simulink model "rfdac_lo_jitter_link_budget"  (R2024a)
settings: Solver=FixedStepDiscrete  StartTime=0.0  StopTime=p.Stop_Time  FixedStep=p.Frame_Period  RelTol=1e-3
PostLoadFcn:
  | addpath(fileparts(get_param('rfdac_lo_jitter_link_budget','FileName'))); setup_rfdac_project;
  | update_rfdac_rx_equalizer_model('rfdac_lo_jitter_link_budget');
  | update_rfdac_lo_amplitude_model('rfdac_lo_jitter_link_budget');
InitFcn:
  | rfdac_model_init;
values from neighbouring files (symbols this model uses):
  cfg = rfdac_default_config()    [init_rfdac_identification.m]    (also in init_rfdac_model.m; run_rfdac_simulation.m = evalin('base','cfg'))
  p = evalin('base','p')    [run_rfdac_simulation.m]
Description:
  | RF TX target-EVM calibration, four-phase LO quadrature imbalance and timing jitter.
settings Model: Creator=Admin  LastModifiedBy=Admin
settings DataIOCC: SaveOutput=off  SignalLogging=off  SaveTime=off

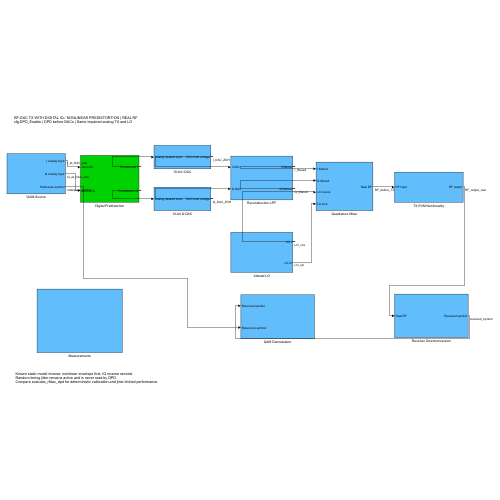
[thumbnail: Simulink's stored preview of the top-level diagram]
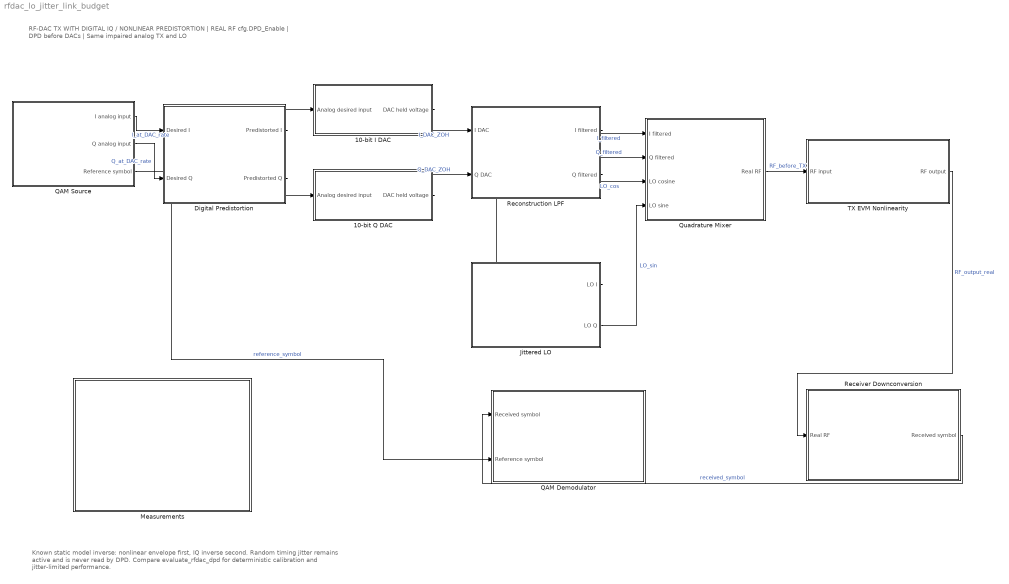
== system rfdac_lo_jitter_link_budget ==
  note: RF-DAC TX WITH DIGITAL IQ / NONLINEAR PREDISTORTION | REAL RF
      | cfg.DPD_Enable | DPD before DACs | Same impaired analog TX and LO
  note: Known static model inverse: nonlinear envelope first, IQ inverse second.
      | Random timing jitter remains active and is never read by DPD.
      | Compare evaluate_rfdac_dpd for deterministic calibration and jitter-limited performance.
  10-bit I DAC : Subsystem
  10-bit Q DAC : Subsystem
  Digital Predistortion : Subsystem  Tag=rfdac_dpd_v7
  Jittered LO : Subsystem
  Measurements : Subsystem
  QAM Demodulator : Subsystem
  QAM Source : Subsystem
  Quadrature Mixer : Subsystem
  Receiver Downconversion : Subsystem
  Reconstruction LPF : Subsystem
  TX EVM Nonlinearity : Subsystem  Tag=rfdac_evm_v2
  wires:
  10-bit I DAC/1(DAC held voltage) -> Reconstruction LPF/1(I DAC)  "I_DAC_ZOH"
  10-bit Q DAC/1(DAC held voltage) -> Reconstruction LPF/2(Q DAC)  "Q_DAC_ZOH"
  Reconstruction LPF/1(I filtered) -> Quadrature Mixer/1(I filtered)  "I_filtered"
  Reconstruction LPF/2(Q filtered) -> Quadrature Mixer/2(Q filtered)  "Q_filtered"
  Jittered LO/1(LO I) -> Quadrature Mixer/3(LO cosine)  "LO_cos"
  Jittered LO/2(LO Q) -> Quadrature Mixer/4(LO sine)  "LO_sin"
  Quadrature Mixer/1(Real RF) -> TX EVM Nonlinearity/1(RF input)  "RF_before_TX"
  TX EVM Nonlinearity/1(RF output) -> Receiver Downconversion/1(Real RF)  "RF_output_real"
  Receiver Downconversion/1(Received symbol) -> QAM Demodulator/1(Received symbol)  "received_symbol"
  QAM Source/3(Reference symbol) -> QAM Demodulator/2(Reference symbol)  "reference_symbol"
  QAM Source/1(I analog input) -> Digital Predistortion/1(Desired I)  "I_at_DAC_rate"
  QAM Source/2(Q analog input) -> Digital Predistortion/2(Desired Q)  "Q_at_DAC_rate"
  Digital Predistortion/1(Predistorted I) -> 10-bit I DAC/1(Analog desired input)
  Digital Predistortion/2(Predistorted Q) -> 10-bit Q DAC/1(Analog desired input)

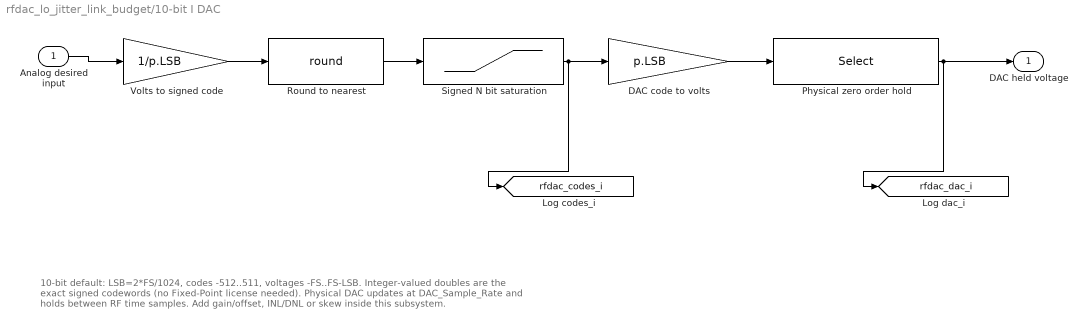
== system rfdac_lo_jitter_link_budget/10-bit I DAC ==
  note: 10-bit default: LSB=2*FS/1024, codes -512..511, voltages -FS..FS-LSB.
      | Integer-valued doubles are the exact signed codewords (no Fixed-Point license needed).
      | Physical DAC updates at DAC_Sample_Rate and holds between RF time samples.
      | Add gain/offset, INL/DNL or skew inside this subsystem.
  Analog desired input : Inport
  DAC code to volts : Gain  Gain=p.LSB
  Physical zero order hold : Selector  InputPortWidth=p.DAC_Samples_Per_Symbol  IndexOptions=Index vector (dialog)  Indices=p.DAC_Hold_Indices  OutputSizes=1
  Round to nearest : Rounding  Operator=round
  Signed N bit saturation : Saturate  UpperLimit=p.Max_Code  LowerLimit=p.Min_Code
  Volts to signed code : Gain  Gain=1/p.LSB
  DAC held voltage : Outport
  tag scope: rfdac_codes_i=global, rfdac_dac_i=global
  wires:
  Analog desired input/1 -> Volts to signed code/1
  Volts to signed code/1 -> Round to nearest/1
  Round to nearest/1 -> Signed N bit saturation/1
  Signed N bit saturation/1 -> DAC code to volts/1, [rfdac_codes_i]
  DAC code to volts/1 -> Physical zero order hold/1
  Physical zero order hold/1 -> DAC held voltage/1, [rfdac_dac_i]

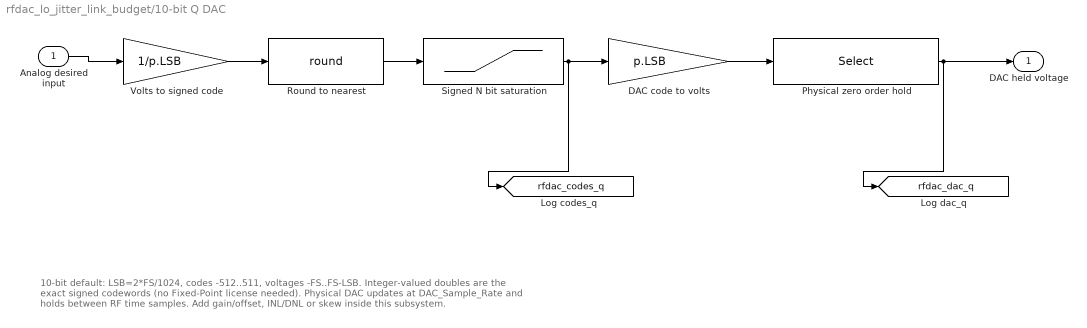
== system rfdac_lo_jitter_link_budget/10-bit Q DAC ==
  note: 10-bit default: LSB=2*FS/1024, codes -512..511, voltages -FS..FS-LSB.
      | Integer-valued doubles are the exact signed codewords (no Fixed-Point license needed).
      | Physical DAC updates at DAC_Sample_Rate and holds between RF time samples.
      | Add gain/offset, INL/DNL or skew inside this subsystem.
  Analog desired input : Inport
  DAC code to volts : Gain  Gain=p.LSB
  Physical zero order hold : Selector  InputPortWidth=p.DAC_Samples_Per_Symbol  IndexOptions=Index vector (dialog)  Indices=p.DAC_Hold_Indices  OutputSizes=1
  Round to nearest : Rounding  Operator=round
  Signed N bit saturation : Saturate  UpperLimit=p.Max_Code  LowerLimit=p.Min_Code
  Volts to signed code : Gain  Gain=1/p.LSB
  DAC held voltage : Outport
  tag scope: rfdac_codes_q=global, rfdac_dac_q=global
  wires:
  Analog desired input/1 -> Volts to signed code/1
  Volts to signed code/1 -> Round to nearest/1
  Round to nearest/1 -> Signed N bit saturation/1
  Signed N bit saturation/1 -> DAC code to volts/1, [rfdac_codes_q]
  DAC code to volts/1 -> Physical zero order hold/1
  Physical zero order hold/1 -> DAC held voltage/1, [rfdac_dac_q]

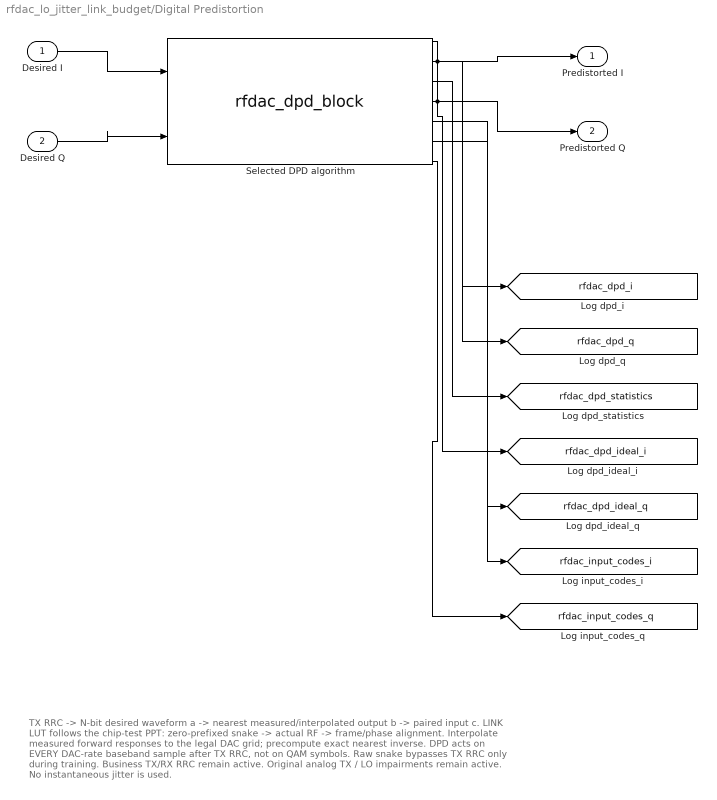
== system rfdac_lo_jitter_link_budget/Digital Predistortion ==
  note: TX RRC -> N-bit desired waveform a -> nearest measured/interpolated output b -> paired input c.
      | LINK LUT follows the chip-test PPT: zero-prefixed snake -> actual RF -> frame/phase alignment.
      | Interpolate measured forward responses to the legal DAC grid; precompute exact nearest inverse.
      | DPD acts on EVERY DAC-rate baseband sample after TX RRC, not on QAM symbols.
      | Raw snake bypasses TX RRC only during training. Business TX/RX RRC remain active.
      | Original analog TX / LO impairments remain active. No instantaneous jitter is used.
  Desired I : Inport
  Desired Q : Inport  Port=2
  Selected DPD algorithm : M-S-Function  FunctionName=rfdac_dpd_block  Parameters=p.DPD_Runtime,p.DAC_Samples_Per_Symbol
  Predistorted I : Outport
  Predistorted Q : Outport  Port=2
  tag scope: rfdac_dpd_i=global, rfdac_dpd_ideal_i=global, rfdac_dpd_ideal_q=global, rfdac_dpd_q=global, rfdac_dpd_statistics=global, rfdac_input_codes_i=global, rfdac_input_codes_q=global
  wires:
  Desired I/1 -> Selected DPD algorithm/1
  Desired Q/1 -> Selected DPD algorithm/2
  Selected DPD algorithm/1 -> Predistorted I/1, [rfdac_dpd_i]
  Selected DPD algorithm/2 -> Predistorted Q/1, [rfdac_dpd_q]
  Selected DPD algorithm/3 -> [rfdac_dpd_statistics]
  Selected DPD algorithm/4 -> [rfdac_dpd_ideal_i]
  Selected DPD algorithm/5 -> [rfdac_dpd_ideal_q]
  Selected DPD algorithm/6 -> [rfdac_input_codes_i]
  Selected DPD algorithm/7 -> [rfdac_input_codes_q]

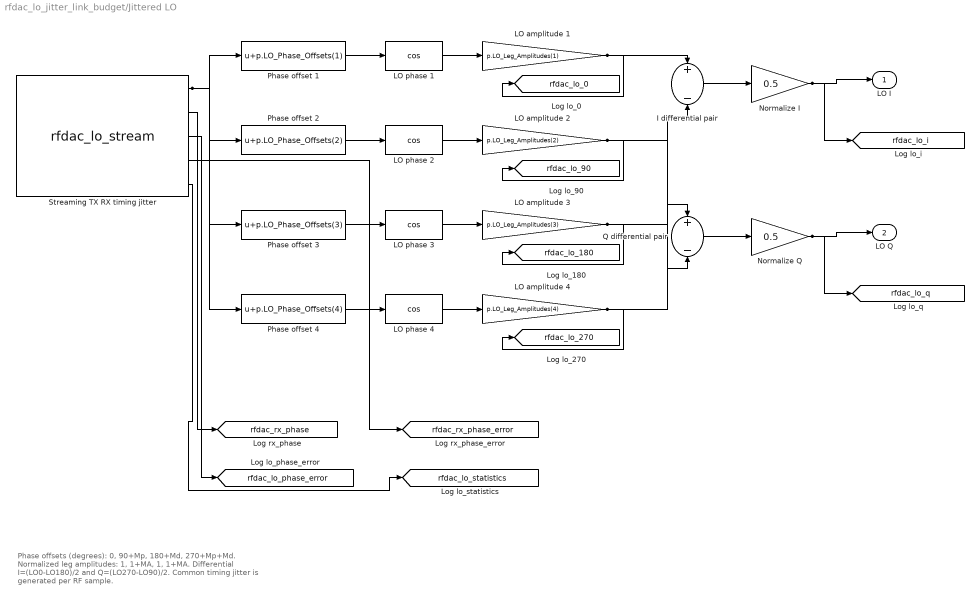
== system rfdac_lo_jitter_link_budget/Jittered LO ==
  note: Phase offsets (degrees): 0, 90+Mp, 180+Md, 270+Mp+Md.
      | Normalized leg amplitudes: 1, 1+MA, 1, 1+MA.
      | Differential I=(LO0-LO180)/2 and Q=(LO270-LO90)/2.
      | Common timing jitter is generated per RF sample.
  I differential pair : Sum  Inputs=+-
  LO amplitude 1 : Gain  Tag=rfdac_lo_leg_amplitude_v1  Gain=p.LO_Leg_Amplitudes(1)
  LO amplitude 2 : Gain  Tag=rfdac_lo_leg_amplitude_v1  Gain=p.LO_Leg_Amplitudes(2)
  LO amplitude 3 : Gain  Tag=rfdac_lo_leg_amplitude_v1  Gain=p.LO_Leg_Amplitudes(3)
  LO amplitude 4 : Gain  Tag=rfdac_lo_leg_amplitude_v1  Gain=p.LO_Leg_Amplitudes(4)
  LO phase {1..4} (4 alike) : Trigonometry  Operator=cos
  Normalize I : Gain  Gain=0.5
  Normalize Q : Gain  Gain=0.5
  Phase offset 1 : Bias  Bias=p.LO_Phase_Offsets(1)  SaturateOnIntegerOverflow=off
  Phase offset 2 : Bias  Bias=p.LO_Phase_Offsets(2)  SaturateOnIntegerOverflow=off
  Phase offset 3 : Bias  Bias=p.LO_Phase_Offsets(3)  SaturateOnIntegerOverflow=off
  Phase offset 4 : Bias  Bias=p.LO_Phase_Offsets(4)  SaturateOnIntegerOverflow=off
  Q differential pair : Sum  Inputs=+-
  Streaming TX RX timing jitter : M-S-Function  FunctionName=rfdac_lo_stream  Parameters=cfg,p.Samples_Per_Symbol
  LO I : Outport
  LO Q : Outport  Port=2
  tag scope: rfdac_lo_0=global, rfdac_lo_180=global, rfdac_lo_270=global, rfdac_lo_90=global, rfdac_lo_i=global, rfdac_lo_phase_error=global, rfdac_lo_q=global, rfdac_lo_statistics=global, rfdac_rx_phase=global, rfdac_rx_phase_error=global
  wires:
  Streaming TX RX timing jitter/1 -> Phase offset 1/1, Phase offset 2/1, Phase offset 3/1, Phase offset 4/1
  Phase offset 1/1 -> LO phase 1/1
  Phase offset 2/1 -> LO phase 2/1
  Phase offset 3/1 -> LO phase 3/1
  Phase offset 4/1 -> LO phase 4/1
  I differential pair/1 -> Normalize I/1
  Q differential pair/1 -> Normalize Q/1
  Normalize I/1 -> LO I/1, [rfdac_lo_i]
  Normalize Q/1 -> LO Q/1, [rfdac_lo_q]
  Streaming TX RX timing jitter/2 -> [rfdac_rx_phase]
  Streaming TX RX timing jitter/3 -> [rfdac_lo_phase_error]
  Streaming TX RX timing jitter/4 -> [rfdac_rx_phase_error]
  Streaming TX RX timing jitter/5 -> [rfdac_lo_statistics]
  LO phase 1/1 -> LO amplitude 1/1
  LO amplitude 1/1 -> [rfdac_lo_0], I differential pair/1
  LO phase 2/1 -> LO amplitude 2/1
  LO amplitude 2/1 -> [rfdac_lo_90], Q differential pair/2
  LO phase 3/1 -> LO amplitude 3/1
  LO amplitude 3/1 -> [rfdac_lo_180], I differential pair/2
  LO phase 4/1 -> LO amplitude 4/1
  LO amplitude 4/1 -> [rfdac_lo_270], Q differential pair/1

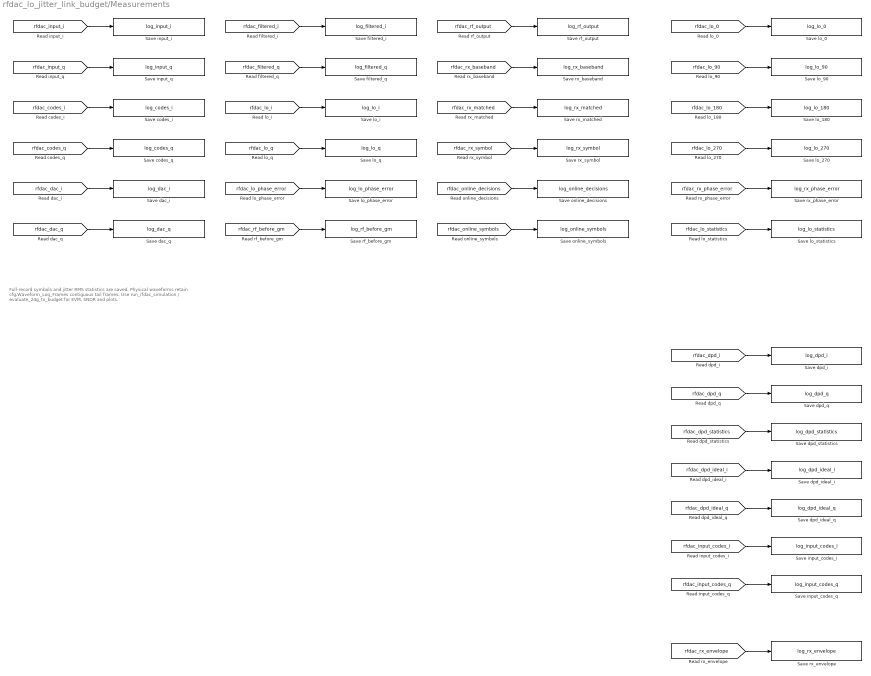
== system rfdac_lo_jitter_link_budget/Measurements ==
  note: Full-record symbols and jitter RMS statistics are saved.
      | Physical waveforms retain cfg.Waveform_Log_Frames contiguous tail frames.
      | Use run_rfdac_simulation / evaluate_24g_tx_budget for EVM, SNDR and plots.
  Save codes_i : ToWorkspace  VariableName=log_codes_i  SaveFormat=Structure With Time  SampleTime=-1
      settings: MaxDataPoints=cfg.Waveform_Log_Frames
  Save codes_q : ToWorkspace  VariableName=log_codes_q  SaveFormat=Structure With Time  SampleTime=-1
      settings: MaxDataPoints=cfg.Waveform_Log_Frames
  Save dac_i : ToWorkspace  VariableName=log_dac_i  SaveFormat=Structure With Time  SampleTime=-1
      settings: MaxDataPoints=cfg.Waveform_Log_Frames
  Save dac_q : ToWorkspace  VariableName=log_dac_q  SaveFormat=Structure With Time  SampleTime=-1
      settings: MaxDataPoints=cfg.Waveform_Log_Frames
  Save dpd_i : ToWorkspace  VariableName=log_dpd_i  SaveFormat=Structure With Time  SampleTime=-1
      settings: MaxDataPoints=cfg.Waveform_Log_Frames
  Save dpd_ideal_i : ToWorkspace  VariableName=log_dpd_ideal_i  SaveFormat=Structure With Time  SampleTime=-1
      settings: MaxDataPoints=cfg.Waveform_Log_Frames
  Save dpd_ideal_q : ToWorkspace  VariableName=log_dpd_ideal_q  SaveFormat=Structure With Time  SampleTime=-1
      settings: MaxDataPoints=cfg.Waveform_Log_Frames
  Save dpd_q : ToWorkspace  VariableName=log_dpd_q  SaveFormat=Structure With Time  SampleTime=-1
      settings: MaxDataPoints=cfg.Waveform_Log_Frames
  Save dpd_statistics : ToWorkspace  VariableName=log_dpd_statistics  SaveFormat=Structure With Time  SampleTime=-1
  Save filtered_i : ToWorkspace  VariableName=log_filtered_i  SaveFormat=Structure With Time  SampleTime=-1
      settings: MaxDataPoints=cfg.Waveform_Log_Frames
  Save filtered_q : ToWorkspace  VariableName=log_filtered_q  SaveFormat=Structure With Time  SampleTime=-1
      settings: MaxDataPoints=cfg.Waveform_Log_Frames
  Save input_codes_i : ToWorkspace  VariableName=log_input_codes_i  SaveFormat=Structure With Time  SampleTime=-1
      settings: MaxDataPoints=cfg.Waveform_Log_Frames
  Save input_codes_q : ToWorkspace  VariableName=log_input_codes_q  SaveFormat=Structure With Time  SampleTime=-1
      settings: MaxDataPoints=cfg.Waveform_Log_Frames
  Save input_i : ToWorkspace  VariableName=log_input_i  SaveFormat=Structure With Time  SampleTime=-1
      settings: MaxDataPoints=cfg.Waveform_Log_Frames
  Save input_q : ToWorkspace  VariableName=log_input_q  SaveFormat=Structure With Time  SampleTime=-1
      settings: MaxDataPoints=cfg.Waveform_Log_Frames
  Save lo_0 : ToWorkspace  VariableName=log_lo_0  SaveFormat=Structure With Time  SampleTime=-1
      settings: MaxDataPoints=cfg.Waveform_Log_Frames
  Save lo_180 : ToWorkspace  VariableName=log_lo_180  SaveFormat=Structure With Time  SampleTime=-1
      settings: MaxDataPoints=cfg.Waveform_Log_Frames
  Save lo_270 : ToWorkspace  VariableName=log_lo_270  SaveFormat=Structure With Time  SampleTime=-1
      settings: MaxDataPoints=cfg.Waveform_Log_Frames
  Save lo_90 : ToWorkspace  VariableName=log_lo_90  SaveFormat=Structure With Time  SampleTime=-1
      settings: MaxDataPoints=cfg.Waveform_Log_Frames
  Save lo_i : ToWorkspace  VariableName=log_lo_i  SaveFormat=Structure With Time  SampleTime=-1
      settings: MaxDataPoints=cfg.Waveform_Log_Frames
  Save lo_phase_error : ToWorkspace  VariableName=log_lo_phase_error  SaveFormat=Structure With Time  SampleTime=-1
      settings: MaxDataPoints=cfg.Waveform_Log_Frames
  Save lo_q : ToWorkspace  VariableName=log_lo_q  SaveFormat=Structure With Time  SampleTime=-1
      settings: MaxDataPoints=cfg.Waveform_Log_Frames
  Save lo_statistics : ToWorkspace  VariableName=log_lo_statistics  SaveFormat=Structure With Time  SampleTime=-1
  Save online_decisions : ToWorkspace  VariableName=log_online_decisions  SaveFormat=Structure With Time  SampleTime=-1
  Save online_symbols : ToWorkspace  VariableName=log_online_symbols  SaveFormat=Structure With Time  SampleTime=-1
  Save rf_before_gm : ToWorkspace  VariableName=log_rf_before_gm  SaveFormat=Structure With Time  SampleTime=-1
      settings: MaxDataPoints=cfg.Waveform_Log_Frames
  Save rf_output : ToWorkspace  VariableName=log_rf_output  SaveFormat=Structure With Time  SampleTime=-1
      settings: MaxDataPoints=cfg.Waveform_Log_Frames
  Save rx_baseband : ToWorkspace  VariableName=log_rx_baseband  SaveFormat=Structure With Time  SampleTime=-1
      settings: MaxDataPoints=cfg.Waveform_Log_Frames
  Save rx_envelope : ToWorkspace  VariableName=log_rx_envelope  SaveFormat=Structure With Time  SampleTime=-1
      settings: MaxDataPoints=p.Observation_Log_Frames
  Save rx_matched : ToWorkspace  VariableName=log_rx_matched  SaveFormat=Structure With Time  SampleTime=-1
      settings: MaxDataPoints=cfg.Waveform_Log_Frames
  Save rx_phase_error : ToWorkspace  VariableName=log_rx_phase_error  SaveFormat=Structure With Time  SampleTime=-1
      settings: MaxDataPoints=cfg.Waveform_Log_Frames
  Save rx_symbol : ToWorkspace  VariableName=log_rx_symbol  SaveFormat=Structure With Time  SampleTime=-1
  wires:
  [rfdac_input_i] -> Save input_i/1
  [rfdac_input_q] -> Save input_q/1
  [rfdac_codes_i] -> Save codes_i/1
  [rfdac_codes_q] -> Save codes_q/1
  [rfdac_dac_i] -> Save dac_i/1
  [rfdac_dac_q] -> Save dac_q/1
  [rfdac_filtered_i] -> Save filtered_i/1
  [rfdac_filtered_q] -> Save filtered_q/1
  [rfdac_lo_i] -> Save lo_i/1
  [rfdac_lo_q] -> Save lo_q/1
  [rfdac_lo_phase_error] -> Save lo_phase_error/1
  [rfdac_rf_before_gm] -> Save rf_before_gm/1
  [rfdac_rf_output] -> Save rf_output/1
  [rfdac_rx_baseband] -> Save rx_baseband/1
  [rfdac_rx_matched] -> Save rx_matched/1
  [rfdac_rx_symbol] -> Save rx_symbol/1
  [rfdac_online_decisions] -> Save online_decisions/1
  [rfdac_online_symbols] -> Save online_symbols/1
  [rfdac_lo_0] -> Save lo_0/1
  [rfdac_lo_90] -> Save lo_90/1
  [rfdac_lo_180] -> Save lo_180/1
  [rfdac_lo_270] -> Save lo_270/1
  [rfdac_rx_phase_error] -> Save rx_phase_error/1
  [rfdac_lo_statistics] -> Save lo_statistics/1
  [rfdac_dpd_i] -> Save dpd_i/1
  [rfdac_dpd_q] -> Save dpd_q/1
  [rfdac_dpd_statistics] -> Save dpd_statistics/1
  [rfdac_dpd_ideal_i] -> Save dpd_ideal_i/1
  [rfdac_dpd_ideal_q] -> Save dpd_ideal_q/1
  [rfdac_input_codes_i] -> Save input_codes_i/1
  [rfdac_input_codes_q] -> Save input_codes_q/1
  [rfdac_rx_envelope] -> Save rx_envelope/1

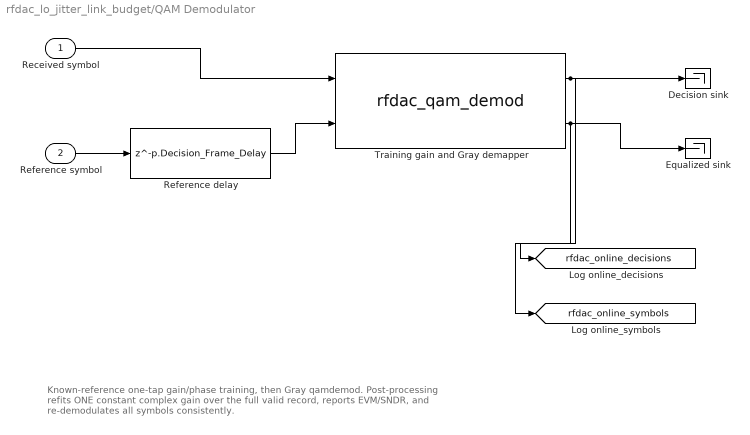
== system rfdac_lo_jitter_link_budget/QAM Demodulator ==
  note: Known-reference one-tap gain/phase training, then Gray qamdemod.
      | Post-processing refits ONE constant complex gain over the full valid record,
      | reports EVM/SNDR, and re-demodulates all symbols consistently.
  Received symbol : Inport
  Reference symbol : Inport  Port=2
  Decision sink : Terminator
  Equalized sink : Terminator
  Reference delay : Delay  DelayLength=p.Decision_Frame_Delay
  Training gain and Gray demapper : M-S-Function  FunctionName=rfdac_qam_demod  Parameters=cfg.QAM_Order
  tag scope: rfdac_online_decisions=global, rfdac_online_symbols=global
  wires:
  Received symbol/1 -> Training gain and Gray demapper/1
  Reference symbol/1 -> Reference delay/1
  Reference delay/1 -> Training gain and Gray demapper/2
  Training gain and Gray demapper/1 -> Decision sink/1, [rfdac_online_decisions]
  Training gain and Gray demapper/2 -> Equalized sink/1, [rfdac_online_symbols]

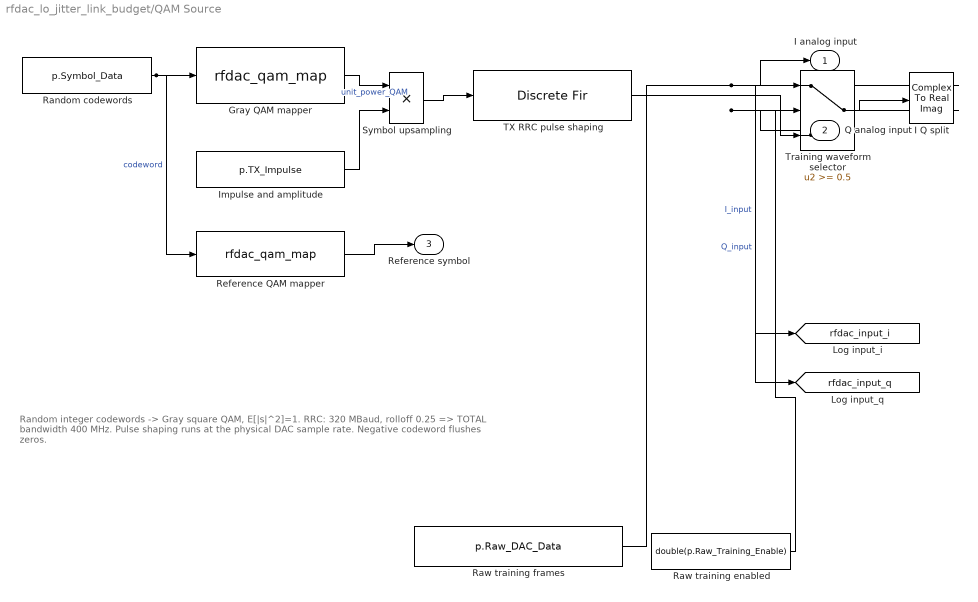
== system rfdac_lo_jitter_link_budget/QAM Source ==
  note: Random integer codewords -> Gray square QAM, E[|s|^2]=1.
      | RRC: 320 MBaud, rolloff 0.25 => TOTAL bandwidth 400 MHz.
      | Pulse shaping runs at the physical DAC sample rate. Negative codeword flushes zeros.
  Gray QAM mapper : M-S-Function  FunctionName=rfdac_qam_map  Parameters=p.Source_Constellation
  I Q split : ComplexToRealImag
  Impulse and amplitude : Constant  Value=p.TX_Impulse
  Random codewords : FromWorkspace  VariableName=p.Symbol_Data  SampleTime=p.Frame_Period  Interpolate=off  OutputAfterFinalValue=Holding final value
  Raw training enabled : Constant  Value=double(p.Raw_Training_Enable)
  Raw training frames : FromWorkspace  VariableName=p.Raw_DAC_Data  SampleTime=p.Frame_Period  Interpolate=off  OutputAfterFinalValue=Holding final value
  Reference QAM mapper : M-S-Function  FunctionName=rfdac_qam_map  Parameters=p.Constellation
  Symbol upsampling : Product
  TX RRC pulse shaping : DiscreteFir  Coefficients=p.RRC  InputProcessing=Columns as channels (frame based)
  Training waveform selector : Switch  Threshold=0.5  SaturateOnIntegerOverflow=off  InputSameDT=off
  I analog input : Outport
  Q analog input : Outport  Port=2
  Reference symbol : Outport  Port=3
  tag scope: rfdac_input_i=global, rfdac_input_q=global
  wires:
  Random codewords/1 -> Gray QAM mapper/1, Reference QAM mapper/1  "codeword"
  Gray QAM mapper/1 -> Symbol upsampling/1  "unit_power_QAM"
  Impulse and amplitude/1 -> Symbol upsampling/2
  Symbol upsampling/1 -> TX RRC pulse shaping/1
  I Q split/1 -> I analog input/1, [rfdac_input_i]  "I_input"
  I Q split/2 -> Q analog input/1, [rfdac_input_q]  "Q_input"
  Reference QAM mapper/1 -> Reference symbol/1
  Raw training frames/1 -> Training waveform selector/1
  Raw training enabled/1 -> Training waveform selector/2
  TX RRC pulse shaping/1 -> Training waveform selector/3
  Training waveform selector/1 -> I Q split/1

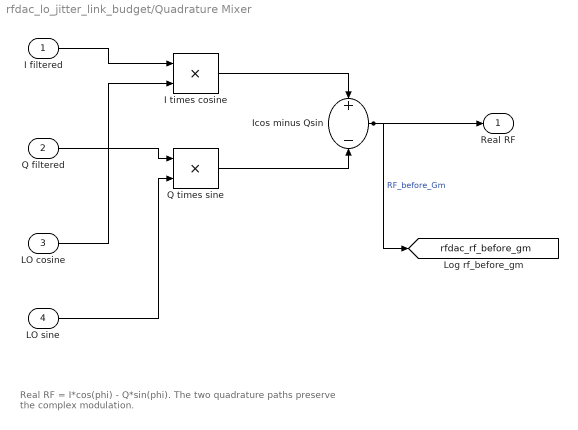
== system rfdac_lo_jitter_link_budget/Quadrature Mixer ==
  note: Real RF = I*cos(phi) - Q*sin(phi).
      | The two quadrature paths preserve the complex modulation.
  I filtered : Inport
  Q filtered : Inport  Port=2
  LO cosine : Inport  Port=3
  LO sine : Inport  Port=4
  I times cosine : Product
  Icos minus Qsin : Sum  Inputs=+-
  Q times sine : Product
  Real RF : Outport
  tag scope: rfdac_rf_before_gm=global
  wires:
  I filtered/1 -> I times cosine/1
  LO cosine/1 -> I times cosine/2
  Q filtered/1 -> Q times sine/1
  LO sine/1 -> Q times sine/2
  I times cosine/1 -> Icos minus Qsin/1
  Q times sine/1 -> Icos minus Qsin/2
  Icos minus Qsin/1 -> Real RF/1, [rfdac_rf_before_gm]  "RF_before_Gm"

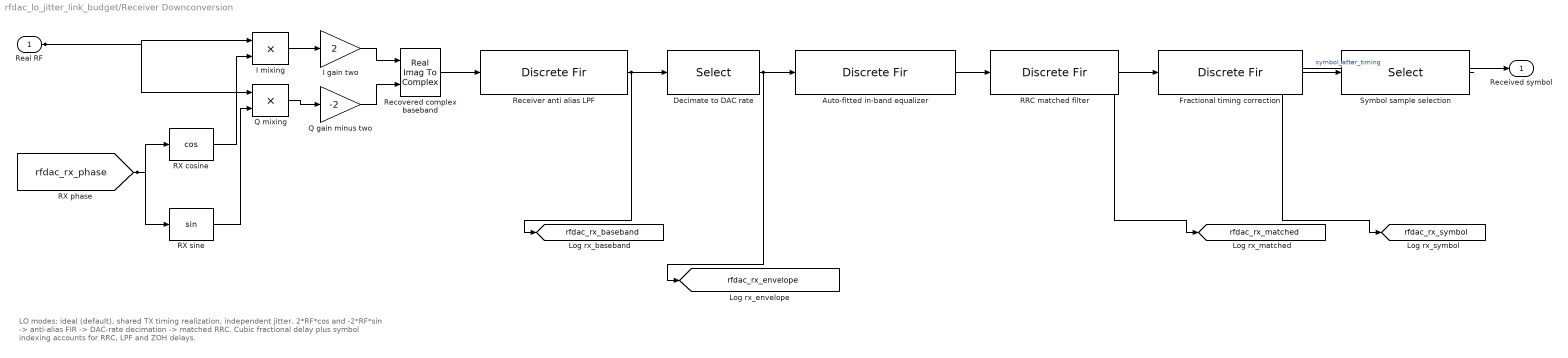
== system rfdac_lo_jitter_link_budget/Receiver Downconversion ==
  note: LO modes: ideal (default), shared TX timing realization, independent jitter.
      | 2*RF*cos and -2*RF*sin -> anti-alias FIR -> DAC-rate decimation -> matched RRC.
      | Cubic fractional delay plus symbol indexing accounts for RRC, LPF and ZOH delays.
  Real RF : Inport
  Auto-fitted in-band equalizer : DiscreteFir  Tag=rfdac_rx_equalizer_v1  Description=|  Coefficients=p.RX_Equalizer_FIR  InputProcessing=Columns as channels (frame based)
      | Causal FIR fitted automatically to the configured TX/RX LPF responses.
      | Runs at DAC_Sample_Rate before the RRC matched filter.
      | cfg.RX_Equalizer_Enable=false selects the unity coefficient.
      | Its known FIR delay is included in receive symbol/reference timing.
  Decimate to DAC rate : Selector  InputPortWidth=p.Samples_Per_Symbol  IndexOptions=Index vector (dialog)  Indices=p.RX_Decimation_Indices  OutputSizes=1
  Fractional timing correction : DiscreteFir  Coefficients=p.Fractional_FIR  InputProcessing=Columns as channels (frame based)
  I gain two : Gain  Gain=2
  I mixing : Product
  Q gain minus two : Gain  Gain=-2
  Q mixing : Product
  RRC matched filter : DiscreteFir  Coefficients=p.RX_RRC  InputProcessing=Columns as channels (frame based)
  RX cosine : Trigonometry  Operator=cos
  RX sine : Trigonometry
  Receiver anti alias LPF : DiscreteFir  Coefficients=p.RX_FIR  InputProcessing=Columns as channels (frame based)
  Recovered complex baseband : RealImagToComplex
  Symbol sample selection : Selector  InputPortWidth=p.DAC_Samples_Per_Symbol  IndexOptions=Index vector (dialog)  Indices=p.Decision_Index  OutputSizes=1
  Received symbol : Outport
  tag scope: rfdac_rx_baseband=global, rfdac_rx_envelope=global, rfdac_rx_matched=global, rfdac_rx_symbol=global
  wires:
  Real RF/1 -> I mixing/1, Q mixing/1
  RX cosine/1 -> I mixing/2
  RX sine/1 -> Q mixing/2
  I mixing/1 -> I gain two/1
  Q mixing/1 -> Q gain minus two/1
  I gain two/1 -> Recovered complex baseband/1
  Q gain minus two/1 -> Recovered complex baseband/2
  Recovered complex baseband/1 -> Receiver anti alias LPF/1
  Receiver anti alias LPF/1 -> Decimate to DAC rate/1, [rfdac_rx_baseband]
  Decimate to DAC rate/1 -> [rfdac_rx_envelope], Auto-fitted in-band equalizer/1
  RRC matched filter/1 -> Fractional timing correction/1
  Fractional timing correction/1 -> Symbol sample selection/1, [rfdac_rx_matched]
  Symbol sample selection/1 -> Received symbol/1, [rfdac_rx_symbol]  "symbol_after_timing"
  [rfdac_rx_phase] -> RX cosine/1, RX sine/1
  Auto-fitted in-band equalizer/1 -> RRC matched filter/1

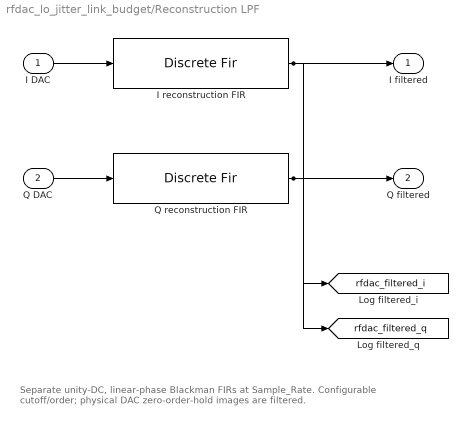
== system rfdac_lo_jitter_link_budget/Reconstruction LPF ==
  note: Separate unity-DC, linear-phase Blackman FIRs at Sample_Rate.
      | Configurable cutoff/order; physical DAC zero-order-hold images are filtered.
  I DAC : Inport
  Q DAC : Inport  Port=2
  I reconstruction FIR : DiscreteFir  Coefficients=p.TX_FIR  InputProcessing=Columns as channels (frame based)
  Q reconstruction FIR : DiscreteFir  Coefficients=p.TX_FIR  InputProcessing=Columns as channels (frame based)
  I filtered : Outport
  Q filtered : Outport  Port=2
  tag scope: rfdac_filtered_i=global, rfdac_filtered_q=global
  wires:
  I DAC/1 -> I reconstruction FIR/1
  Q DAC/1 -> Q reconstruction FIR/1
  I reconstruction FIR/1 -> I filtered/1, [rfdac_filtered_i]
  Q reconstruction FIR/1 -> Q filtered/1, [rfdac_filtered_q]

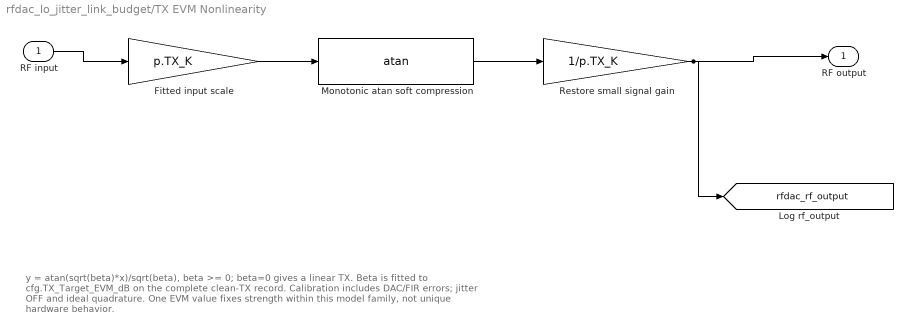
== system rfdac_lo_jitter_link_budget/TX EVM Nonlinearity ==
  note: y = atan(sqrt(beta)*x)/sqrt(beta), beta >= 0; beta=0 gives a linear TX.
      | Beta is fitted to cfg.TX_Target_EVM_dB on the complete clean-TX record.
      | Calibration includes DAC/FIR errors; jitter OFF and ideal quadrature.
      | One EVM value fixes strength within this model family, not unique hardware behavior.
  RF input : Inport
  Fitted input scale : Gain  Gain=p.TX_K
  Monotonic atan soft compression : Trigonometry  Operator=atan
  Restore small signal gain : Gain  Gain=1/p.TX_K
  RF output : Outport
  tag scope: rfdac_rf_output=global
  wires:
  RF input/1 -> Fitted input scale/1
  Fitted input scale/1 -> Monotonic atan soft compression/1
  Monotonic atan soft compression/1 -> Restore small signal gain/1
  Restore small signal gain/1 -> RF output/1, [rfdac_rf_output]
